simulink model "reference_07_divergent_fixed_point"  (R2026b)
settings: Solver=FixedStepDiscrete  StartTime=0  StopTime=0.5  FixedStep=0.01  RelTol=1e-10  AbsTol=1e-12
settings Model: Creator=Fasih  LastModifiedBy=Fasih
settings DataIOCC: SaveOutput=off

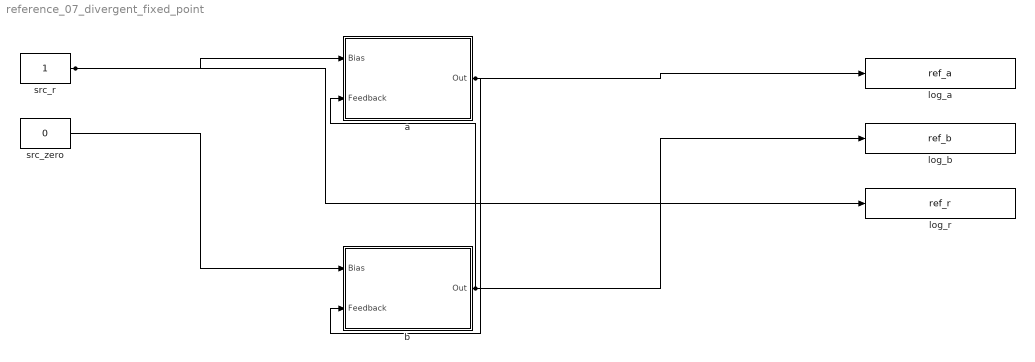
== system reference_07_divergent_fixed_point ==
  a : Subsystem
  b : Subsystem
  log_a : ToWorkspace  VariableName=ref_a  SaveFormat=Timeseries  SampleTime=0.01
  log_b : ToWorkspace  VariableName=ref_b  SaveFormat=Timeseries  SampleTime=0.01
  log_r : ToWorkspace  VariableName=ref_r  SaveFormat=Timeseries  SampleTime=0.01
  src_r : Constant  OutDataTypeStr=double
  src_zero : Constant  Value=0  OutDataTypeStr=double
  wires:
  src_r/1 -> a/1(Bias), log_r/1
  src_zero/1 -> b/1(Bias)
  b/1(Out) -> a/2(Feedback), log_b/1
  a/1(Out) -> b/2(Feedback), log_a/1

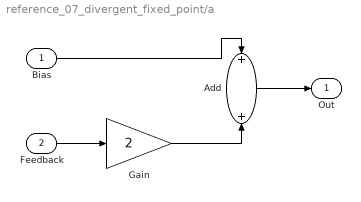
== system reference_07_divergent_fixed_point/a ==
  Bias : Inport
  Feedback : Inport  Port=2
  Add : Sum
  Gain : Gain  Gain=2
  Out : Outport
  wires:
  Bias/1 -> Add/1
  Feedback/1 -> Gain/1
  Gain/1 -> Add/2
  Add/1 -> Out/1

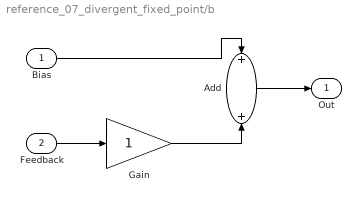
== system reference_07_divergent_fixed_point/b ==
  Bias : Inport
  Feedback : Inport  Port=2
  Add : Sum
  Gain : Gain
  Out : Outport
  wires:
  Bias/1 -> Add/1
  Feedback/1 -> Gain/1
  Gain/1 -> Add/2
  Add/1 -> Out/1
